simulink model "ball_balance_sim"  (R2026b)
settings: Solver=daessc  StopTime=bb.Tsim  MaxStep=1e-3
PreLoadFcn:
  | addpath(fileparts(which(bdroot))); bb = bb_params();
InitFcn:
  | addpath(fileparts(which(bdroot))); bb = bb_params();
values from neighbouring files (symbols this model uses):
  bb = bb_params();',      'Solver', 'daessc', 'StopTime', stopTime, 'MaxStep', '1e-3',      'RelTol', '1e-3', 'SaveOutput', 'on', 'SaveFormat', 'Dataset',      'ReturnWorkspaceOutputs', 'on', 'SignalLogging', 'on')    [build_bb_model.m]    (also in design_controller.m = bb_params(); run_closed_loop.m = bb_params(); run_open_loop_test.m = bb_params())
  deg = 90    [build_bb_model.m]
  kg = blk(C, 'simulink/Math Operations/Gain', 'LQI Gain', [860 100])    [build_bb_model.m]
  s = @(t0, T) min(max((t - t0)/T, 0), 1)    [bb_params.m]    (also in run_open_loop_test.m = squeeze(srv.Data); if size(s,1) == 2 && size(s,2) ~= 2, s = )
undefined symbols (not defined in the file or in its folder): X, Y, Z
libraries: sm_lib x54, nesl_utility x9
(part 1 of 2)
settings Model: Creator=PC  LastModifiedBy=PC
settings SimscapeCC: SimscapeLogType=all  SimscapeNominalValues="[{\"value\":\"1\",\"unit\":\"A\"},{\"value\":\"1\",\"unit\":\"bar\"},{\"value\":\"1\",\"unit\":\"cm^2\"},{\"value\":\"1\",\"unit\":\"cm^3/s\"},{\"value\":\"1\",\"unit\":\"kJ/kg\"},{\"value\":\"1\",\"unit\":\"kW\"},{\"value\":\"1\",\"unit\":\"l\"},{\"value\":\"1\",\"unit\":\"N\"},{\"value\":\"1\",\"unit\":\"N*m\"},{\"value\":\"1\",\"unit\":\"V\"},{\"value\":\"0.001\",\"unit\":\"Wb\"}]"  SimscapeUseEnergyAccounting=off

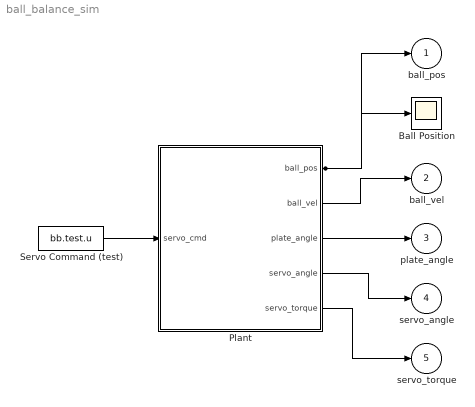
== system ball_balance_sim ==
  Ball Position : Scope
  Plant : Subsystem
  Servo Command (test) : FromWorkspace  VariableName=bb.test.u  Interpolate=off  OutputAfterFinalValue=Holding final value
  ball_pos : Outport
  ball_vel : Outport  Port=2
  plate_angle : Outport  Port=3
  servo_angle : Outport  Port=4
  servo_torque : Outport  Port=5
  wires:
  Plant/1(ball_pos) -> ball_pos/1, Ball Position/1
  Servo Command (test)/1 -> Plant/1(servo_cmd)
  Plant/2(ball_vel) -> ball_vel/1
  Plant/3(plate_angle) -> plate_angle/1
  Plant/4(servo_angle) -> servo_angle/1
  Plant/5(servo_torque) -> servo_torque/1
